simulink model "testing"  (R2025b)
settings: Solver=FixedStepDiscrete  StartTime=0.0  StopTime=20  RelTol=1e-3
InitFcn:
  | mcb_pmsm_foc_qep_f28379d_SIUnit_data
values from neighbouring files (symbols this model uses):
  A = [ -Rs/L,           0,                  0 ... (first row only)    [mcb_pmsm_fsfb_f28379d_param.m]    (also in v0_pmsm_fsfb_sim_for_flipsky_.m = [; v1_0_3_sim_param_fsfc.m = [)
  inverter = mcb.updateInverterParameters(pmsm,inverter,target)    [mcb_pmsm_foc_qep_f28379d_SIUnit_data.m]
  K = Ka_fsfb(1)    [mcb_pmsm_foc_qep_f28379d_SIUnit_data.m]    (also in mcb_pmsm_fsfb_f28379d_param.m = place(Ai, Bi, desired_poles); v0_pmsm_fsfb_sim_for_flipsky_.m = place(Ai, Bi, desired_poles); v1_0_3_sim_param_fsfc.m = place(Ai, Bi, desired_poles))
  Ki = -Ka_fsfb(2)    [mcb_pmsm_foc_qep_f28379d_SIUnit_data.m]    (also in mcb_pmsm_fsfb_f28379d_param.m = -K(:, n+1:end); v0_pmsm_fsfb_sim_for_flipsky_.m = -K(:, n+1:end); v1_0_3_sim_param_fsfc.m = -K(:, n+1:end))
  lambda_pm = pmsm.FluxPM    [mcb_pmsm_foc_qep_f28379d_SIUnit_data.m]
  PI_params = mcb.calcFOCGains(motor,Ts,Ts_speed,SpdLPFltCoeff=LPFltCoeff)    [mcb_pmsm_foc_qep_f28379d_SIUnit_data.m]
  pmsm = mcb.getPMSMParameters('Teknic2310P')    [mcb_pmsm_foc_qep_f28379d_SIUnit_data.m]
  Speed_Ki_Ts = Kis * Ts_speed    [mcb_pmsm_foc_qep_f28379d_SIUnit_data.m]
  Speed_Kp = Ks    [mcb_pmsm_foc_qep_f28379d_SIUnit_data.m]
  T_pwm = 1/PWM_frequency    (= 5e-05)    [mcb_pmsm_foc_qep_f28379d_SIUnit_data.m]
  target = mcb.getProcessorParameters('F28379D',PWM_frequency)    [mcb_pmsm_foc_qep_f28379d_SIUnit_data.m]
  Ts = T_pwm    (= 5e-05)    [mcb_pmsm_foc_qep_f28379d_SIUnit_data.m]    (also in v0_pmsm_fsfb_sim_for_flipsky_.m = 0.0001; v1_0_3_sim_param_fsfc.m = 0.0001)
  Ts_inverter = T_pwm/2    (= 2.5e-05)    [mcb_pmsm_foc_qep_f28379d_SIUnit_data.m]
  Ts_motor = T_pwm/2    (= 2.5e-05)    [mcb_pmsm_foc_qep_f28379d_SIUnit_data.m]
  Ts_simulink = T_pwm/2    (= 2.5e-05)    [mcb_pmsm_foc_qep_f28379d_SIUnit_data.m]
  Ts_speed = 10*Ts    (= 0.0005)    [mcb_pmsm_foc_qep_f28379d_SIUnit_data.m]
undefined symbols (not defined in the file or in its folder): bit, DiscIntNeverNeededParam, Down, GPTRIP1SEL, GPTRIP2SEL, TZ1, TZ2, Up
libraries: mcbcontrolslib x10, c2802xlib x7, simulink x5, c2837xDlib x4, mcbeeMathTransformLib x3, c280xlib x3, mcbpositiondecoderlib x3, svdschedulerlib x1, autolibpmsmexterior x1, slpidlib x1
(part 2 of 2)

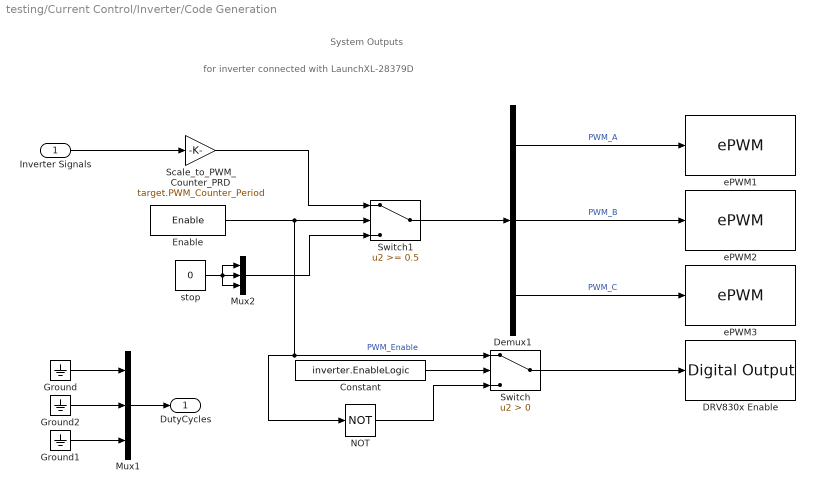
== system testing/Current Control/Inverter/Code Generation ==
  note: for inverter connected with LaunchXL-28379D
  note: System Outputs
  Inverter Signals : Inport
  Constant : Constant  Value=inverter.EnableLogic
  DRV830x Enable : c2837xDlib/Digital Output  GPIO_Number=GPIO120~GPIO127  GPIO_Bit0=off  GPIO_BIT0_Toggle=off  GPIO_Bit1=off  GPIO_BIT1_Toggle=off  GPIO_Bit2=off  GPIO_BIT2_Toggle=off  GPIO_Bit3=off  GPIO_BIT3_Toggle=off  GPIO_Bit4=on  GPIO_BIT4_Toggle=off  GPIO_Bit5=off  GPIO_BIT5_Toggle=off  GPIO_Bit6=off  GPIO_BIT6_Toggle=off  GPIO_Bit7=off  GPIO_BIT7_Toggle=off
  Demux1 : Demux  Outputs=3
  Enable : DataStoreRead  DataStoreName=Enable  IndexOptions=Index vector (dialog)  Indices=1  OutputSizes=1
  Ground : Ground
  Ground1 : Ground
  Ground2 : Ground
  Mux1 : Mux  Inputs=3
  Mux2 : Mux  Inputs=3
  NOT : Logic  Operator=NOT  IconShape=distinctive  AllPortsSameDT=off  OutDataTypeStr=boolean
  Scale_to_PWM_Counter_PRD : Gain  Gain=target.PWM_Counter_Period  OutDataTypeStr=uint16  RndMeth=Simplest
  Switch : Switch  Criteria=u2 > Threshold  SaturateOnIntegerOverflow=off  InputSameDT=off
  Switch1 : Switch  Threshold=0.5  SaturateOnIntegerOverflow=off  InputSameDT=off
  ePWM1 : c2802xlib/ePWM  PwmType=C2000_Type4  useModule=ePWM1  ePWMxLINKTBPRD=Not Linked  periodUnits=Clock cycles  timerSource=Specify via dialog  timerPeriod_clk=target.PWM_Counter_Period  timerPeriod_sec=0.0001  tbshadow=Counter equals to zero  countingMode=Up-Down  phaseActiveEnable=Disable  phaseDirection=Count down after sync  phaseActive=0  synchronizationEnable=off  dcaevt1Sync=off  dcbevt1Sync=off  synchronizationOption=Counter equals to zero (CTR=Zero)  dcbevt1SyncOut=off  dcaevt1SyncOut=off  cmpdSyncOut=off  cmpcSyncOut=off  cmpbSyncOut=off  zeroSyncOut=on  swfSyncOut=off  perSynchronizationOption=Counter equals to period (CTR=PRD)  clockPrescale=1  HSclockPrescale=1  enswap=off  ePWMxAStatus=on  ePWMxAactionLogic1=Do nothing  ePWMxAactionLogic2=Do nothing  ePWMxAactionLogic3=Clear  ePWMxAactionLogic4=Set  ePWMxAactionLogic5=Do nothing  ePWMxAactionLogic6=Do nothing  ePWMxACSFenable=off  ePWMxACSFvalue=Forcing disable  ePWMxASFreload=Zero  ePWMxBStatus=off  ePWMxBactionLogic1=Set  ePWMxBactionLogic2=Clear  ePWMxBactionLogic3=Do nothing  ePWMxBactionLogic4=Do nothing  ePWMxBactionLogic5=Clear  ePWMxBactionLogic6=Set  ePWMxBCSFenable=off  ePWMxBCSFvalue=Forcing disable  ePWMxBSFreload=Zero  ePWNxBOutWay=off  ePWMxLINKCMPA=Not Linked  CMPAUnits=Clock cycles  CMPASource=Input port  CMPAValue_per=50  CMPAValue_clk=floor(target.PWM_Counter_Period/2+1)  enCMPAshadow=Counter equals to zero (CTR=Zero)  ePWMxLINKCMPB=Not Linked  CMPBUnits=Clock cycles  CMPBSource=Specify via dialog  CMPBValue_per=50  CMPBValue_clk=floor(target.PWM_Counter_Period/2+1)  enCMPBshadow=Counter equals to zero (CTR=Zero)  ePWMxLINKCMPC=Not Linked  CMPCUnits=Clock cycles  CMPCSource=Specify via dialog  CMPCValue_per=50  CMPCValue_clk=32000  enCMPCshadow=Counter equals to zero (CTR=Zero)  ePWMxLINKCMPD=Not Linked  CMPDUnits=Clock cycles  CMPDSource=Specify via dialog  CMPDValue_per=50  CMPDValue_clk=32000  enCMPDshadow=Counter equals to zero (CTR=Zero)  enableDBePWMxA=on  enableDBePWMxB=on  enhalfcycle=off  DBpolarity=Active high complementary (AHC)  DBedgeDelay=Positive  DBSource_ePWMxA=ePWMxA  DBSource_ePWMxB=ePWMxA  DBPeriodUnits=Clock cycles  DBperiodSource=Specify via dialog  REDperiod=15  FEDperiod=15  REDperiod_sec=0  FEDperiod_sec=0  LoadModeDBRED=Immediate without using shadow  LoadModeDBFED=Immediate without using shadow  adcstartModuleA=on  adcrequestEventA=First event  adcstartEventA=Digital Compare Module A Event 1 start of conversion (DCAEVT1.soc)  adcstartEventA_type2=Counter equals to period (CTR=PRD)  adcstartModuleB=off  adcrequestEventB=First event  adcstartEventB=Counter equals to zero (CTR=Zero)  adcstartEventB_type2=Counter equals to zero (CTR=Zero)  intEn=off  intPrd=First event  intSel=Counter equals to zero (CTR=Zero)  intSel_type2=Counter equals to zero (CTR=Zero)  hrpe=off  enHRPWM=off  HRPWM_LoadMode=Counter equals to period (CTR=PRD)  HRPWM_CTLMode=Duty or Period control mode  HRPWM_EDGMode=Both edge  hrpeb=off  enHRPWMB=off  HRPWM_LoadModeB=Counter equals to zero (CTR=ZERO)  HRPWM_CTLModeB=Duty or Period control mode  HRPWM_EDGModeB=Both edge  enHRDBRED=off  enHRDBFED=off  enSFO=on  enautoconv=on  chopperEnable=off  chopperFrequency=1  chopperFirstwidth=1  chopperDuty=12.5%  tripZonesource=Specify via dialog  tzselOSHT1=off  tzselOSHT2=off  tzselOSHT3=off  tzselOSHT4=off  tzselOSHT5=off  tzselOSHT6=off  tzselOSHDCAEV1=off  tzselOSHDCBEV1=off  tzselCBC1=off  tzselCBC2=off  tzselCBC3=off  tzselCBC4=off  tzselCBC5=off  tzselCBC6=off  tzselCBCDCAEV2=off  tzselCBCDCBEV2=off  enTzOstIntr=off  enTzCbcIntr=off  enTzDCAEVT1Intr=off  enTzDCAEVT2Intr=off  enTzDCBEVT1Intr=off  enTzDCBEVT2Intr=off  tzclrCBCLatch=Counter equals to zero (CTR=Zero)  ePWMxAforced=No action  ePWMxBforced=No action  DCAEVT1forced=No action  DCBEVT1forced=No action  DCAEVT2forced=No action  DCBEVT2forced=No action  dcah=Trip Zone 1 input (TZ1)  dcal=Trip Zone 2 input (TZ2)  dcbh=Trip Zone 1 input (TZ1)  dcbl=Trip Zone 2 input (TZ2)  dcah_type2=GPTRIP1SEL/(TZ1)  dcal_type2=GPTRIP2SEL/(TZ2)  dcbh_type2=GPTRIP1SEL/(TZ1)  dcbl_type2=GPTRIP2SEL/(TZ2)  gendcaevt1=Event disabled  gendcaevt2=Event disabled  gendcbevt1=Event disabled  gendcbevt2=Event disabled  dcaevt1src=DCAEVT1 with sync  dcaevt2src=DCAEVT2 with sync  dcbevt1src=DCBEVT1 with sync  dcbevt2src=DCBEVT2 with sync  pulsesel=Counter equals to zero (CTR=Zero)  blankinv=off  blankoffset=0  blankwidth=0  evsrcsel=Filtered version of DCAEVT1 (DCAEVT1FILT)  encape=off
  ePWM2 : c2802xlib/ePWM  PwmType=C2000_Type4  useModule=ePWM2  ePWMxLINKTBPRD=Not Linked  periodUnits=Clock cycles  timerSource=Specify via dialog  timerPeriod_clk=target.PWM_Counter_Period  timerPeriod_sec=0.0001  tbshadow=Counter equals to zero  countingMode=Up-Down  phaseActiveEnable=Set counter to phase value specified via dialog  phaseDirection=Count up after sync  phaseActive=0  synchronizationEnable=off  dcaevt1Sync=off  dcbevt1Sync=off  synchronizationOption=Pass through (EPWMxSYNCI or SWFSYNC)  dcbevt1SyncOut=off  dcaevt1SyncOut=off  cmpdSyncOut=off  cmpcSyncOut=off  cmpbSyncOut=off  zeroSyncOut=off  swfSyncOut=on  perSynchronizationOption=Counter equals to period (CTR=PRD)  clockPrescale=1  HSclockPrescale=1  enswap=off  ePWMxAStatus=on  ePWMxAactionLogic1=Do nothing  ePWMxAactionLogic2=Do nothing  ePWMxAactionLogic3=Clear  ePWMxAactionLogic4=Set  ePWMxAactionLogic5=Do nothing  ePWMxAactionLogic6=Do nothing  ePWMxACSFenable=off  ePWMxACSFvalue=Forcing disable  ePWMxASFreload=Zero  ePWMxBStatus=off  ePWMxBactionLogic1=Set  ePWMxBactionLogic2=Clear  ePWMxBactionLogic3=Do nothing  ePWMxBactionLogic4=Do nothing  ePWMxBactionLogic5=Clear  ePWMxBactionLogic6=Set  ePWMxBCSFenable=off  ePWMxBCSFvalue=Forcing disable  ePWMxBSFreload=Zero  ePWNxBOutWay=off  ePWMxLINKCMPA=Not Linked  CMPAUnits=Clock cycles  CMPASource=Input port  CMPAValue_per=50  CMPAValue_clk=floor(target.PWM_Counter_Period/2+1)  enCMPAshadow=Counter equals to zero (CTR=Zero)  ePWMxLINKCMPB=Not Linked  CMPBUnits=Clock cycles  CMPBSource=Specify via dialog  CMPBValue_per=50  CMPBValue_clk=floor(target.PWM_Counter_Period/2+1)  enCMPBshadow=Counter equals to zero (CTR=Zero)  ePWMxLINKCMPC=Not Linked  CMPCUnits=Clock cycles  CMPCSource=Specify via dialog  CMPCValue_per=50  CMPCValue_clk=32000  enCMPCshadow=Counter equals to zero (CTR=Zero)  ePWMxLINKCMPD=Not Linked  CMPDUnits=Clock cycles  CMPDSource=Specify via dialog  CMPDValue_per=50  CMPDValue_clk=32000  enCMPDshadow=Counter equals to zero (CTR=Zero)  enableDBePWMxA=on  enableDBePWMxB=on  enhalfcycle=off  DBpolarity=Active high complementary (AHC)  DBedgeDelay=Positive  DBSource_ePWMxA=ePWMxA  DBSource_ePWMxB=ePWMxA  DBPeriodUnits=Clock cycles  DBperiodSource=Specify via dialog  REDperiod=15  FEDperiod=15  REDperiod_sec=0  FEDperiod_sec=0  LoadModeDBRED=Immediate without using shadow  LoadModeDBFED=Immediate without using shadow  adcstartModuleA=off  adcrequestEventA=First event  adcstartEventA=Digital Compare Module A Event 1 start of conversion (DCAEVT1.soc)  adcstartEventA_type2=Counter equals to period (CTR=PRD)  adcstartModuleB=off  adcrequestEventB=First event  adcstartEventB=Counter equals to zero (CTR=Zero)  adcstartEventB_type2=Counter equals to zero (CTR=Zero)  intEn=off  intPrd=First event  intSel=Counter equals to zero (CTR=Zero)  intSel_type2=Counter equals to zero (CTR=Zero)  hrpe=off  enHRPWM=off  HRPWM_LoadMode=Counter equals to period (CTR=PRD)  HRPWM_CTLMode=Duty or Period control mode  HRPWM_EDGMode=Both edge  hrpeb=off  enHRPWMB=off  HRPWM_LoadModeB=Counter equals to zero (CTR=ZERO)  HRPWM_CTLModeB=Duty or Period control mode  HRPWM_EDGModeB=Both edge  enHRDBRED=off  enHRDBFED=off  enSFO=on  enautoconv=on  chopperEnable=off  chopperFrequency=1  chopperFirstwidth=1  chopperDuty=12.5%  tripZonesource=Specify via dialog  tzselOSHT1=off  tzselOSHT2=off  tzselOSHT3=off  tzselOSHT4=off  tzselOSHT5=off  tzselOSHT6=off  tzselOSHDCAEV1=off  tzselOSHDCBEV1=off  tzselCBC1=off  tzselCBC2=off  tzselCBC3=off  tzselCBC4=off  tzselCBC5=off  tzselCBC6=off  tzselCBCDCAEV2=off  tzselCBCDCBEV2=off  enTzOstIntr=off  enTzCbcIntr=off  enTzDCAEVT1Intr=off  enTzDCAEVT2Intr=off  enTzDCBEVT1Intr=off  enTzDCBEVT2Intr=off  tzclrCBCLatch=Counter equals to zero (CTR=Zero)  ePWMxAforced=No action  ePWMxBforced=No action  DCAEVT1forced=No action  DCBEVT1forced=No action  DCAEVT2forced=No action  DCBEVT2forced=No action  dcah=Trip Zone 1 input (TZ1)  dcal=Trip Zone 2 input (TZ2)  dcbh=Trip Zone 1 input (TZ1)  dcbl=Trip Zone 2 input (TZ2)  dcah_type2=GPTRIP1SEL/(TZ1)  dcal_type2=GPTRIP2SEL/(TZ2)  dcbh_type2=GPTRIP1SEL/(TZ1)  dcbl_type2=GPTRIP2SEL/(TZ2)  gendcaevt1=Event disabled  gendcaevt2=Event disabled  gendcbevt1=Event disabled  gendcbevt2=Event disabled  dcaevt1src=DCAEVT1 with sync  dcaevt2src=DCAEVT2 with sync  dcbevt1src=DCBEVT1 with sync  dcbevt2src=DCBEVT2 with sync  pulsesel=Counter equals to zero (CTR=Zero)  blankinv=off  blankoffset=0  blankwidth=0  evsrcsel=Filtered version of DCAEVT1 (DCAEVT1FILT)  encape=off
  ePWM3 : c2802xlib/ePWM  PwmType=C2000_Type4  useModule=ePWM3  ePWMxLINKTBPRD=Not Linked  periodUnits=Clock cycles  timerSource=Specify via dialog  timerPeriod_clk=target.PWM_Counter_Period  timerPeriod_sec=0.0001  tbshadow=Counter equals to zero  countingMode=Up-Down  phaseActiveEnable=Set counter to phase value specified via dialog  phaseDirection=Count up after sync  phaseActive=0  synchronizationEnable=off  dcaevt1Sync=off  dcbevt1Sync=off  synchronizationOption=Pass through (EPWMxSYNCI or SWFSYNC)  dcbevt1SyncOut=off  dcaevt1SyncOut=off  cmpdSyncOut=off  cmpcSyncOut=off  cmpbSyncOut=off  zeroSyncOut=off  swfSyncOut=on  perSynchronizationOption=Counter equals to period (CTR=PRD)  clockPrescale=1  HSclockPrescale=1  enswap=off  ePWMxAStatus=on  ePWMxAactionLogic1=Do nothing  ePWMxAactionLogic2=Do nothing  ePWMxAactionLogic3=Clear  ePWMxAactionLogic4=Set  ePWMxAactionLogic5=Do nothing  ePWMxAactionLogic6=Do nothing  ePWMxACSFenable=off  ePWMxACSFvalue=Forcing disable  ePWMxASFreload=Zero  ePWMxBStatus=off  ePWMxBactionLogic1=Set  ePWMxBactionLogic2=Clear  ePWMxBactionLogic3=Do nothing  ePWMxBactionLogic4=Do nothing  ePWMxBactionLogic5=Clear  ePWMxBactionLogic6=Set  ePWMxBCSFenable=off  ePWMxBCSFvalue=Forcing disable  ePWMxBSFreload=Zero  ePWNxBOutWay=off  ePWMxLINKCMPA=Not Linked  CMPAUnits=Clock cycles  CMPASource=Input port  CMPAValue_per=50  CMPAValue_clk=floor(target.PWM_Counter_Period/2+1)  enCMPAshadow=Counter equals to zero (CTR=Zero)  ePWMxLINKCMPB=Not Linked  CMPBUnits=Clock cycles  CMPBSource=Specify via dialog  CMPBValue_per=50  CMPBValue_clk=floor(target.PWM_Counter_Period/2+1)  enCMPBshadow=Counter equals to zero (CTR=Zero)  ePWMxLINKCMPC=Not Linked  CMPCUnits=Clock cycles  CMPCSource=Specify via dialog  CMPCValue_per=50  CMPCValue_clk=32000  enCMPCshadow=Counter equals to zero (CTR=Zero)  ePWMxLINKCMPD=Not Linked  CMPDUnits=Clock cycles  CMPDSource=Specify via dialog  CMPDValue_per=50  CMPDValue_clk=32000  enCMPDshadow=Counter equals to zero (CTR=Zero)  enableDBePWMxA=on  enableDBePWMxB=on  enhalfcycle=off  DBpolarity=Active high complementary (AHC)  DBedgeDelay=Positive  DBSource_ePWMxA=ePWMxA  DBSource_ePWMxB=ePWMxA  DBPeriodUnits=Clock cycles  DBperiodSource=Specify via dialog  REDperiod=15  FEDperiod=15  REDperiod_sec=0  FEDperiod_sec=0  LoadModeDBRED=Immediate without using shadow  LoadModeDBFED=Immediate without using shadow  adcstartModuleA=off  adcrequestEventA=First event  adcstartEventA=Digital Compare Module A Event 1 start of conversion (DCAEVT1.soc)  adcstartEventA_type2=Counter equals to period (CTR=PRD)  adcstartModuleB=off  adcrequestEventB=First event  adcstartEventB=Counter equals to zero (CTR=Zero)  adcstartEventB_type2=Counter equals to zero (CTR=Zero)  intEn=off  intPrd=First event  intSel=Counter equals to zero (CTR=Zero)  intSel_type2=Counter equals to zero (CTR=Zero)  hrpe=off  enHRPWM=off  HRPWM_LoadMode=Counter equals to period (CTR=PRD)  HRPWM_CTLMode=Duty or Period control mode  HRPWM_EDGMode=Both edge  hrpeb=off  enHRPWMB=off  HRPWM_LoadModeB=Counter equals to zero (CTR=ZERO)  HRPWM_CTLModeB=Duty or Period control mode  HRPWM_EDGModeB=Both edge  enHRDBRED=off  enHRDBFED=off  enSFO=on  enautoconv=on  chopperEnable=off  chopperFrequency=1  chopperFirstwidth=1  chopperDuty=12.5%  tripZonesource=Specify via dialog  tzselOSHT1=off  tzselOSHT2=off  tzselOSHT3=off  tzselOSHT4=off  tzselOSHT5=off  tzselOSHT6=off  tzselOSHDCAEV1=off  tzselOSHDCBEV1=off  tzselCBC1=off  tzselCBC2=off  tzselCBC3=off  tzselCBC4=off  tzselCBC5=off  tzselCBC6=off  tzselCBCDCAEV2=off  tzselCBCDCBEV2=off  enTzOstIntr=off  enTzCbcIntr=off  enTzDCAEVT1Intr=off  enTzDCAEVT2Intr=off  enTzDCBEVT1Intr=off  enTzDCBEVT2Intr=off  tzclrCBCLatch=Counter equals to zero (CTR=Zero)  ePWMxAforced=No action  ePWMxBforced=No action  DCAEVT1forced=No action  DCBEVT1forced=No action  DCAEVT2forced=No action  DCBEVT2forced=No action  dcah=Trip Zone 1 input (TZ1)  dcal=Trip Zone 2 input (TZ2)  dcbh=Trip Zone 1 input (TZ1)  dcbl=Trip Zone 2 input (TZ2)  dcah_type2=GPTRIP1SEL/(TZ1)  dcal_type2=GPTRIP2SEL/(TZ2)  dcbh_type2=GPTRIP1SEL/(TZ1)  dcbl_type2=GPTRIP2SEL/(TZ2)  gendcaevt1=Event disabled  gendcaevt2=Event disabled  gendcbevt1=Event disabled  gendcbevt2=Event disabled  dcaevt1src=DCAEVT1 with sync  dcaevt2src=DCAEVT2 with sync  dcbevt1src=DCBEVT1 with sync  dcbevt2src=DCBEVT2 with sync  pulsesel=Counter equals to zero (CTR=Zero)  blankinv=off  blankoffset=0  blankwidth=0  evsrcsel=Filtered version of DCAEVT1 (DCAEVT1FILT)  encape=off
  stop : Constant  Value=0  OutDataTypeStr=uint16
  DutyCycles : Outport  VectorParamsAs1DForOutWhenUnconnected=off
  wires:
  Demux1/3 -> ePWM3/1  "PWM_C"
  Scale_to_PWM_Counter_PRD/1 -> Switch1/1
  Mux2/1 -> Switch1/3
  stop/1 -> Mux2/3, Mux2/2, Mux2/1
  Enable/1 -> NOT/1, Switch/1, Switch1/2  "PWM_Enable"
  Demux1/2 -> ePWM2/1  "PWM_B"
  Switch1/1 -> Demux1/1
  Demux1/1 -> ePWM1/1  "PWM_A"
  Inverter Signals/1 -> Scale_to_PWM_Counter_PRD/1
  Ground/1 -> Mux1/1
  Ground1/1 -> Mux1/3
  Ground2/1 -> Mux1/2
  Mux1/1 -> DutyCycles/1
  Switch/1 -> DRV830x Enable/1
  NOT/1 -> Switch/3
  Constant/1 -> Switch/2

== system testing/Current Control/Inverter/Simulation ==
  Inverter Signals : Inport
  Data Type Duplicate : DataTypeDuplicate
  Enable : DataStoreRead  DataStoreName=Enable  IndexOptions=Index vector (dialog)  Indices=1  OutputSizes=1
  Mux2 : Mux  Inputs=3
  Switch1 : Switch  Threshold=0.5  RndMeth=Simplest  SaturateOnIntegerOverflow=off  InputSameDT=off
  stop : Constant  Value=0  OutDataTypeStr=Inherit: Inherit via back propagation
  DutyCycles : Outport  VectorParamsAs1DForOutWhenUnconnected=off
  wires:
  stop/1 -> Data Type Duplicate/2, Mux2/1, Mux2/3, Mux2/2
  Mux2/1 -> Switch1/3
  Switch1/1 -> DutyCycles/1
  Inverter Signals/1 -> Data Type Duplicate/1, Switch1/1  "PWM Duty Cycles"
  Enable/1 -> Switch1/2  "PWM_Enable"

== system testing/Hardware Init/Variant Subsystem/Code Generation ==
  note: for BoostXL-DRV8305 connected to LaunchXL-28379D
  note: System Outputs
  note: Enable ADC offset calibration only when motor is not loaded and not rotating due to external factors
  In1 : Inport
  ADC Calibration Enable : Constant  Value=inverter.ADCOffsetCalibEnable
  "Calculate ADC Offset " : Subsystem  Priority=1001  TreatAsAtomicUnit=on
  DRV Enable : Subsystem  Priority=1
  Default ADC Offset : Subsystem  Priority=1001  TreatAsAtomicUnit=on
  NOT : Logic  Operator=NOT  IconShape=distinctive  AllPortsSameDT=off  OutDataTypeStr=boolean
  wires:
  In1/1 -> DRV Enable/1(In)
  NOT/1 -> Default ADC Offset/Enable
  ADC Calibration Enable/1 -> NOT/1, "Calculate ADC Offset "/Enable

== system testing/Hardware Init/Variant Subsystem/Simulation ==
  In1 : Inport
  Terminator : Terminator
  wires:
  In1/1 -> Terminator/1

== system testing/Heartbeat LED/Heartbeat LED/Code generation ==
  In1 : Inport
  Digital Output : c2837xDlib/Digital Output  GPIO_Number=GPIO32~GPIO39  GPIO_Bit0=off  GPIO_BIT0_Toggle=on  GPIO_Bit1=off  GPIO_BIT1_Toggle=off  GPIO_Bit2=on  GPIO_BIT2_Toggle=on  GPIO_Bit3=off  GPIO_BIT3_Toggle=off  GPIO_Bit4=off  GPIO_BIT4_Toggle=off  GPIO_Bit5=off  GPIO_BIT5_Toggle=off  GPIO_Bit6=off  GPIO_BIT6_Toggle=off  GPIO_Bit7=off  GPIO_BIT7_Toggle=off
  wires:
  In1/1 -> Digital Output/1

== system testing/Heartbeat LED/Heartbeat LED/Simulation ==
  In1 : Inport
  Simulation_Terminator : Terminator
  wires:
  In1/1 -> Simulation_Terminator/1

== system testing/Inverter and Motor - Plant Model/Simulation/Inverter ==
  Duty_abc : Inport
  Average_Value_Inverter : Subsystem
  Constant2 : Constant  Value=inverter.V_dc  OutDataTypeStr=single  SampleTime=-1
  Data Type Conversion1 : DataTypeConversion  OutDataTypeStr=single  RndMeth=Simplest  SaturateOnIntegerOverflow=off
  Demux : Demux  Outputs=3
  Inverter_delay : DiscreteTransferFcn  Numerator=[1-exp(-Ts_inverter/(T_pwm/2))]  Denominator=[1 -exp(-Ts_inverter/(T_pwm/2))]  RndMeth=Simplest
  Mux : Mux  Inputs=3
  Rate Transition3 : RateTransition  Integrity=off  OutPortSampleTime=Ts_inverter
  Vabc : Outport  VectorParamsAs1DForOutWhenUnconnected=off
  wires:
  Average_Value_Inverter/2(Vb) -> Mux/2
  Mux/1 -> Inverter_delay/1
  Constant2/1 -> Average_Value_Inverter/4(Vdc)
  Average_Value_Inverter/3(Vc) -> Mux/3
  Average_Value_Inverter/1(Va) -> Mux/1
  Demux/1 -> Average_Value_Inverter/1(Vao)
  Demux/3 -> Average_Value_Inverter/3(Vco)
  Demux/2 -> Average_Value_Inverter/2(Vbo)
  Data Type Conversion1/1 -> Rate Transition3/1
  Rate Transition3/1 -> Demux/1
  Inverter_delay/1 -> Vabc/1
  Duty_abc/1 -> Data Type Conversion1/1

== system testing/Inverter and Motor - Plant Model/Simulation/Load_Profile (Torque) ==
  Data Type Conversion : DataTypeConversion  OutDataTypeStr=single  SaturateOnIntegerOverflow=off  RndMeth=Floor
  IIR Filter : mcbcontrolslib/IIR Filter  VariantControl=Low Pass Filter  VariantSelect=Low-pass  FilterConstantInputType=Specify via dialog  Filter_constant=0.01  InitialOutput=Specify via dialog  InitialOutputValue=0  ExternalReset=none  advancedSettings=off  Ts=50e-6  cutOff_freq=32.1525
  T_load : Step  Time=2  Before=0.05*pmsm.T_rated  After=0.5*pmsm.T_rated  SampleTime=Ts_simulink
  Load_Trq : Outport  VectorParamsAs1DForOutWhenUnconnected=off
  wires:
  Data Type Conversion/1 -> IIR Filter/1
  T_load/1 -> Data Type Conversion/1
  IIR Filter/1 -> Load_Trq/1

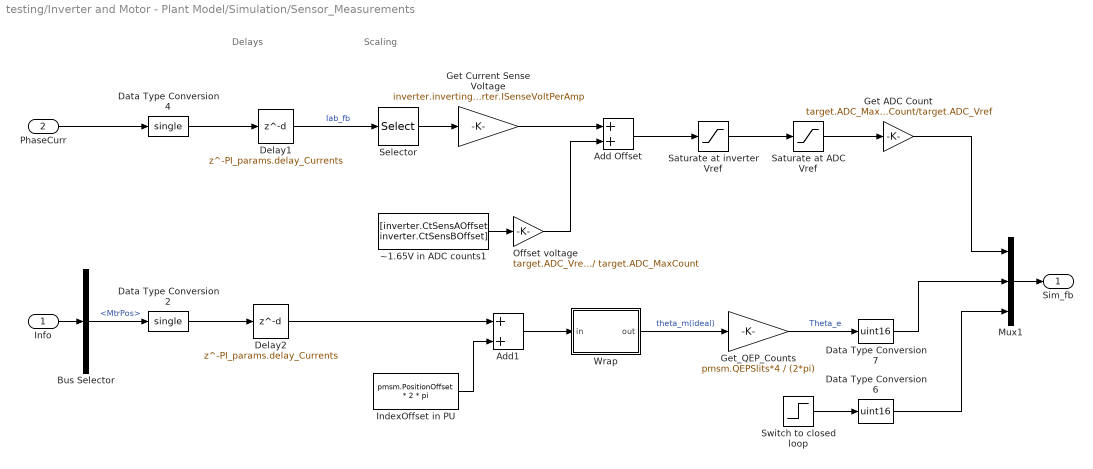
== system testing/Inverter and Motor - Plant Model/Simulation/Sensor_Measurements ==
  note: Scaling
  note: Delays
  Info : Inport
  PhaseCurr : Inport  Port=2
  Add Offset : Sum  RndMeth=Simplest
  Add1 : Sum  RndMeth=Simplest
  Bus Selector : BusSelector  OutputSignals=MtrPos
  Data Type Conversion2 : DataTypeConversion  OutDataTypeStr=single  RndMeth=Simplest  SaturateOnIntegerOverflow=off
  Data Type Conversion4 : DataTypeConversion  OutDataTypeStr=single  RndMeth=Simplest  SaturateOnIntegerOverflow=off
  Data Type Conversion6 : DataTypeConversion  OutDataTypeStr=uint16  RndMeth=Simplest  SaturateOnIntegerOverflow=off
  Data Type Conversion7 : DataTypeConversion  OutDataTypeStr=uint16  RndMeth=Simplest  SaturateOnIntegerOverflow=off
  Delay1 : Delay  DelayLength=PI_params.delay_Currents
  Delay2 : Delay  DelayLength=PI_params.delay_Currents
  Get ADC Count : Gain  Gain=target.ADC_MaxCount/target.ADC_Vref  OutMin=0  OutMax=target.ADC_MaxCount  OutDataTypeStr=uint16  RndMeth=Simplest
  Get Current Sense Voltage : Gain  Gain=inverter.invertingAmp * inverter.ISenseVoltPerAmp  RndMeth=Simplest  OutDataTypeStr=Inherit: Same as input
  Get_QEP_Counts : Gain  Gain=pmsm.QEPSlits*4 / (2*pi)  OutDataTypeStr=uint16  RndMeth=Simplest
  IndexOffset in PU : Constant  Value=pmsm.PositionOffset * 2 * pi  OutDataTypeStr=single  SampleTime=-1
  Mux1 : Mux  Inputs=3
  Offset voltage : Gain  Gain=target.ADC_Vref / target.ADC_MaxCount  RndMeth=Simplest
  Saturate at ADC Vref : Saturate  UpperLimit=target.ADC_Vref  LowerLimit=0
  Saturate at inverter Vref : Saturate  UpperLimit=inverter.ISenseVref  LowerLimit=0
  Selector : Selector  InputPortWidth=3  IndexOptions=Index vector (dialog)  Indices=[1 2]  OutputSizes=1
  Switch to closed loop : Step  Time=0.1  SampleTime=Ts_motor
  Wrap : Subsystem
  ~1.65V in ADC counts1 : Constant  Value=[inverter.CtSensAOffset inverter.CtSensBOffset]  OutDataTypeStr=uint16  SampleTime=-1
  Sim_fb : Outport  VectorParamsAs1DForOutWhenUnconnected=off
  wires:
  Delay1/1 -> Selector/1  "Iab_fb"
  Data Type Conversion4/1 -> Delay1/1
  PhaseCurr/1 -> Data Type Conversion4/1
  Info/1 -> Bus Selector/1
  Bus Selector/1 -> Data Type Conversion2/1  "<MtrPos>"
  Data Type Conversion2/1 -> Delay2/1
  Mux1/1 -> Sim_fb/1
  Delay2/1 -> Add1/1
  IndexOffset in PU/1 -> Add1/2
  Add1/1 -> Wrap/1(in)
  Get_QEP_Counts/1 -> Data Type Conversion7/1  "Theta_e"
  Wrap/1(out) -> Get_QEP_Counts/1  "theta_m(ideal)"
  Switch to closed loop/1 -> Data Type Conversion6/1
  ~1.65V in ADC counts1/1 -> Offset voltage/1
  Get Current Sense Voltage/1 -> Add Offset/1
  Saturate at ADC Vref/1 -> Get ADC Count/1
  Add Offset/1 -> Saturate at inverter Vref/1
  Saturate at inverter Vref/1 -> Saturate at ADC Vref/1
  Selector/1 -> Get Current Sense Voltage/1
  Offset voltage/1 -> Add Offset/2
  Data Type Conversion6/1 -> Mux1/3
  Data Type Conversion7/1 -> Mux1/2
  Get ADC Count/1 -> Mux1/1

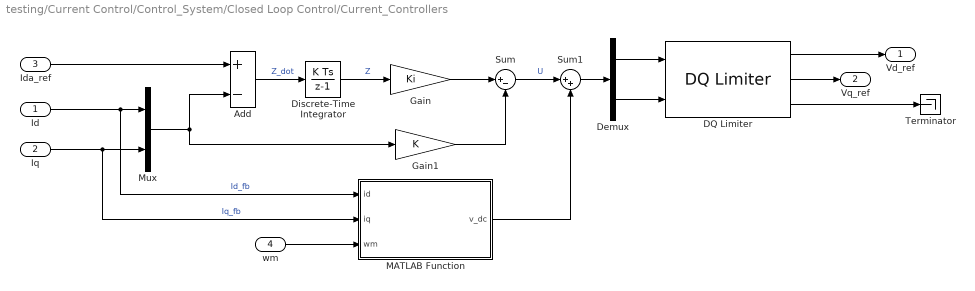
== system testing/Current Control/Control_System/Closed Loop Control/Current_Controllers ==
  Id : Inport
  Iq : Inport  Port=2
  Ida_ref : Inport  Port=3
  wm : Inport  Port=4
  Add : Sum  Inputs=+-
  DQ Limiter : mcbcontrolslib/DQ Limiter  satMethodInputType=Specify via dialog  satMethodSelected=D-Q equivalence  satLimitInputType=Specify via dialog  Vmax=inverter.V_dc/sqrt(3) *0.95
  Demux : Demux  Outputs=2
  Discrete-Time Integrator : DiscreteIntegrator  SampleTime=-1  ICPrevOutput=DiscIntNeverNeededParam  ICPrevScaledInput=DiscIntNeverNeededParam
  Gain : Gain  Gain=Ki
  Gain1 : Gain  Gain=K
  MATLAB Function : MATLAB Function  TreatAsAtomicUnit=on
  Mux : Mux  Inputs=2
  Sum : Sum  Inputs=|+-
  Sum1 : Sum  Inputs=|++
  Terminator : Terminator
  Vd_ref : Outport  VectorParamsAs1DForOutWhenUnconnected=off
  Vq_ref : Outport  Port=2  VectorParamsAs1DForOutWhenUnconnected=off
  wires:
  Ida_ref/1 -> Add/1
  Demux/1 -> DQ Limiter/1
  Demux/2 -> DQ Limiter/2
  DQ Limiter/2 -> Vq_ref/1
  DQ Limiter/1 -> Vd_ref/1
  DQ Limiter/3 -> Terminator/1
  Id/1 -> MATLAB Function/1(id), Mux/1  "Id_fb"
  Iq/1 -> MATLAB Function/2(iq), Mux/2  "Iq_fb"
  Mux/1 -> Gain1/1, Add/2
  Add/1 -> Discrete-Time Integrator/1  "Z_dot"
  Discrete-Time Integrator/1 -> Gain/1  "Z"
  Gain/1 -> Sum/1
  Gain1/1 -> Sum/2
  MATLAB Function/1(v_dc) -> Sum1/2
  Sum/1 -> Sum1/1  "U"
  wm/1 -> MATLAB Function/3(wm)
  Sum1/1 -> Demux/1

== system testing/Current Control/Control_System/Closed Loop Control/SVPWM ==
  Va : Inport
  Vb : Inport  Port=2
  Constant : Constant  Value=0.5  OutDataTypeStr=dataType  SampleTime=-1
  Mux1 : Mux  Inputs=3
  Normalize [-0.5 to 0.5] : Gain  Gain=1/ (2 * inverter.V_dc / sqrt(3))  RndMeth=Simplest  OutDataTypeStr=Inherit: Same as input
  Space Vector Generator : mcbcontrolslib/PWM Reference Generator  inSignal=Valphabeta  modType=SVM: space vector modulation
  Sum : Sum  Inputs=|++
  Duty_abc : Outport
  wires:
  Mux1/1 -> Normalize [-0.5 to 0.5]/1
  Normalize [-0.5 to 0.5]/1 -> Sum/1
  Va/1 -> Space Vector Generator/1
  Space Vector Generator/1 -> Mux1/1
  Constant/1 -> Sum/2
  Space Vector Generator/3 -> Mux1/3
  Space Vector Generator/2 -> Mux1/2
  Vb/1 -> Space Vector Generator/2
  Sum/1 -> Duty_abc/1

== system testing/Current Control/Control_System/Open Loop Start-Up/Convert to Duty Cycles ==
  In : Inport
  Constant : Constant  Value=0.5  OutDataTypeStr=dataType  SampleTime=-1
  Normalize : Gain  Gain=1/2  RndMeth=Simplest  OutDataTypeStr=Inherit: Same as input
  Sum1 : Sum  Inputs=|++
  Out : Outport
  wires:
  Normalize/1 -> Sum1/1
  Constant/1 -> Sum1/2
  In/1 -> Normalize/1
  Sum1/1 -> Out/1

== system testing/Current Control/Control_System/Open Loop Start-Up/Ramp Generator ==
  Ramp_Time : Inport
  Enable : Inport  Port=2
  Divide : Product  Inputs=*/  RndMeth=Simplest  OutDataTypeStr=Inherit: Same as first input
  NOT : Logic  Operator=NOT  IconShape=distinctive  AllPortsSameDT=off  OutDataTypeStr=boolean
  One : Constant  OutDataTypeStr=dataType  SampleTime=-1
  Ramp Generator : DiscreteIntegrator  IntegratorMethod=Accumulation: Forward Euler  gainval=1  ExternalReset=sampled level  SampleTime=-1  OutDataTypeStr=dataType  RndMeth=Simplest  LimitOutput=on  UpperSaturationLimit=1  LowerSaturationLimit=0  ICPrevOutput=DiscIntNeverNeededParam  ICPrevScaledInput=DiscIntNeverNeededParam
  Sample_Time : Gain  Gain=Ts  RndMeth=Simplest  OutDataTypeStr=Inherit: Same as input
  Ramp : Outport
  wires:
  Divide/1 -> Sample_Time/1
  Ramp Generator/1 -> Ramp/1  "Eps"
  Sample_Time/1 -> Ramp Generator/1
  One/1 -> Divide/1
  Ramp_Time/1 -> Divide/2
  Enable/1 -> NOT/1
  NOT/1 -> Ramp Generator/2

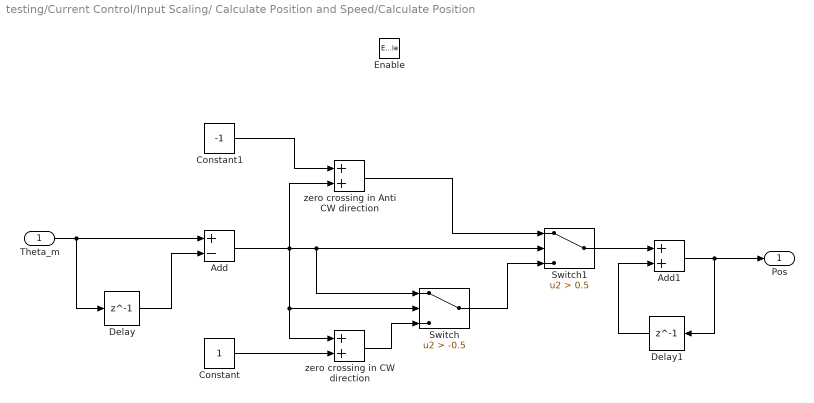
== system testing/Current Control/Input Scaling/ Calculate Position and Speed/Calculate Position ==
  Theta_m : Inport
  Enable : EnablePort
  Add : Sum  Inputs=+-
  Add1 : Sum
  Constant : Constant  OutDataTypeStr=dataType
  Constant1 : Constant  Value=-1  OutDataTypeStr=dataType
  Delay : Delay  DelayLength=1
  Delay1 : Delay  DelayLength=1
  Switch : Switch  Criteria=u2 > Threshold  Threshold=-0.5  SaturateOnIntegerOverflow=off  InputSameDT=off
  Switch1 : Switch  Criteria=u2 > Threshold  Threshold=0.5  SaturateOnIntegerOverflow=off  InputSameDT=off
  zero crossing in Anti CW direction : Sum
  zero crossing in CW direction : Sum
  Pos : Outport
  wires:
  Theta_m/1 -> Delay/1, Add/1
  Delay/1 -> Add/2
  Delay1/1 -> Add1/2
  Add1/1 -> Pos/1, Delay1/1
  Add/1 -> zero crossing in Anti CW direction/2, zero crossing in CW direction/1, Switch/2, Switch/1, Switch1/2
  zero crossing in CW direction/1 -> Switch/3
  Constant1/1 -> zero crossing in Anti CW direction/1
  zero crossing in Anti CW direction/1 -> Switch1/1
  Switch/1 -> Switch1/3
  Switch1/1 -> Add1/1
  Constant/1 -> zero crossing in CW direction/2

== system testing/Current Control/Input Scaling/ Calculate Position and Speed/IndexFinder ==
  In1 : Inport
  Enable : EnablePort
  AND : Logic  AllPortsSameDT=off  OutDataTypeStr=boolean
  Compare To Constant : simulink/Logic and Bit Operations/Compare To Constant  relop===  const=0  OutDataTypeStr=boolean
  Compare To Constant1 : simulink/Logic and Bit Operations/Compare To Constant  relop=>  const=0  OutDataTypeStr=boolean
  Delay3 : Delay  DelayLength=1
  Out1 : Outport
  wires:
  In1/1 -> Delay3/1, Compare To Constant1/1
  Compare To Constant1/1 -> AND/2
  Compare To Constant/1 -> AND/1
  Delay3/1 -> Compare To Constant/1
  AND/1 -> Out1/1

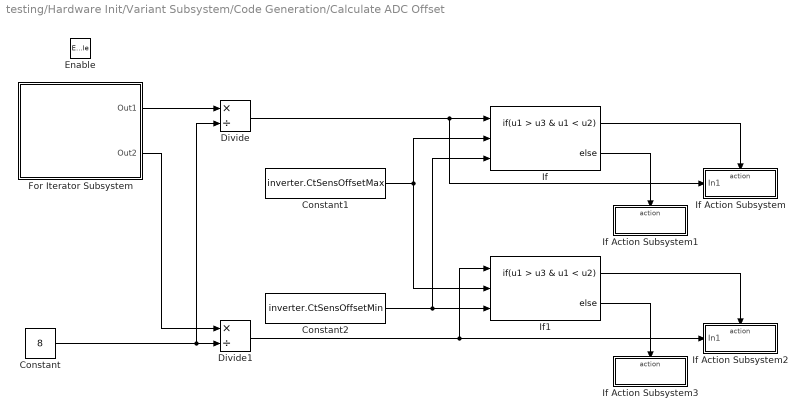
== system testing/Hardware Init/Variant Subsystem/Code Generation/Calculate ADC Offset  ==
  Enable : EnablePort
  Constant : Constant  Value=8
  Constant1 : Constant  Value=inverter.CtSensOffsetMax  OutDataTypeStr=Inherit: Inherit via back propagation
  Constant2 : Constant  Value=inverter.CtSensOffsetMin  OutDataTypeStr=Inherit: Inherit via back propagation
  Divide : Product  Inputs=*/  OutDataTypeStr=uint16
  Divide1 : Product  Inputs=*/  OutDataTypeStr=uint16
  For Iterator Subsystem : Subsystem  TreatAsAtomicUnit=on
  If : If  NumInputs=3  IfExpression=u1 > u3 & u1 < u2
  If Action Subsystem : Subsystem  TreatAsAtomicUnit=on
  If Action Subsystem1 : Subsystem  TreatAsAtomicUnit=on
  If Action Subsystem2 : Subsystem  TreatAsAtomicUnit=on
  If Action Subsystem3 : Subsystem  TreatAsAtomicUnit=on
  If1 : If  NumInputs=3  IfExpression=u1 > u3 & u1 < u2
  wires:
  For Iterator Subsystem/1(Out1) -> Divide/1
  If1/2 -> If Action Subsystem3/Action
  If1/1 -> If Action Subsystem2/Action
  Constant1/1 -> If/2, If1/2
  If/2 -> If Action Subsystem1/Action
  For Iterator Subsystem/2(Out2) -> Divide1/1
  If/1 -> If Action Subsystem/Action
  Constant2/1 -> If/3, If1/3
  Divide1/1 -> If Action Subsystem2/1(In1), If1/1
  Constant/1 -> Divide1/2, Divide/2
  Divide/1 -> If Action Subsystem/1(In1), If/1

== system testing/Hardware Init/Variant Subsystem/Code Generation/DRV Enable ==
  note: Enable Inverter
  In : Inport
  ADC Gain Setting : Subsystem
  Constant : Constant  Value=inverter.EnableLogic
  DRV830x Enable : Constant  OutDataTypeStr=uint16  SampleTime=-1
  Digital Output : c2837xDlib/Digital Output  Priority=10  GPIO_Number=GPIO120~GPIO127  GPIO_Bit0=off  GPIO_BIT0_Toggle=off  GPIO_Bit1=off  GPIO_BIT1_Toggle=off  GPIO_Bit2=off  GPIO_BIT2_Toggle=off  GPIO_Bit3=off  GPIO_BIT3_Toggle=off  GPIO_Bit4=on  GPIO_BIT4_Toggle=off  GPIO_Bit5=off  GPIO_BIT5_Toggle=off  GPIO_Bit6=off  GPIO_BIT6_Toggle=off  GPIO_Bit7=off  GPIO_BIT7_Toggle=off
  Digital Output1 : c2837xDlib/Digital Output  Priority=10  GPIO_Number=GPIO16~GPIO23  GPIO_Bit0=off  GPIO_BIT0_Toggle=off  GPIO_Bit1=off  GPIO_BIT1_Toggle=off  GPIO_Bit2=off  GPIO_BIT2_Toggle=off  GPIO_Bit3=off  GPIO_BIT3_Toggle=off  GPIO_Bit4=off  GPIO_BIT4_Toggle=off  GPIO_Bit5=off  GPIO_BIT5_Toggle=off  GPIO_Bit6=on  GPIO_BIT6_Toggle=off  GPIO_Bit7=off  GPIO_BIT7_Toggle=off
  NOT : Logic  Operator=NOT  IconShape=distinctive  AllPortsSameDT=off  OutDataTypeStr=boolean
  RunTimeMeasurement : Constant  OutDataTypeStr=uint16  SampleTime=-1
  Switch : Switch  Criteria=u2 > Threshold  SaturateOnIntegerOverflow=off  InputSameDT=off
  wires:
  RunTimeMeasurement/1 -> Digital Output1/1
  Switch/1 -> Digital Output/1
  DRV830x Enable/1 -> NOT/1, Switch/1
  NOT/1 -> Switch/3
  Constant/1 -> ADC Gain Setting/Enable, Switch/2
  In/1 -> ADC Gain Setting/1(In)

== system testing/Hardware Init/Variant Subsystem/Code Generation/Default ADC Offset ==
  Enable : EnablePort
  Constant : Constant  Value=inverter.CtSensAOffset  OutDataTypeStr=Inherit: Inherit via back propagation
  Constant1 : Constant  Value=inverter.CtSensBOffset  OutDataTypeStr=Inherit: Inherit via back propagation
  Data Store Write1 : DataStoreWrite  DataStoreName=IaOffset  IndexOptions=Index vector (dialog)  Indices=1  OutputSizes=1
  Data Store Write2 : DataStoreWrite  DataStoreName=IbOffset  IndexOptions=Index vector (dialog)  Indices=1  OutputSizes=1
  wires:
  Constant/1 -> Data Store Write1/1
  Constant1/1 -> Data Store Write2/1

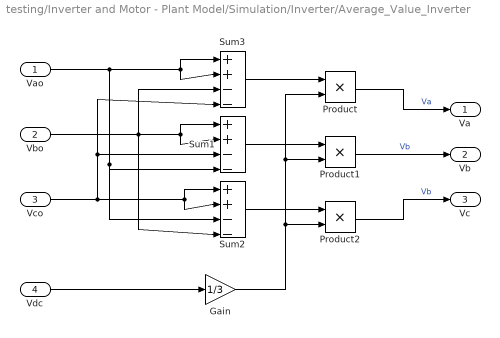
== system testing/Inverter and Motor - Plant Model/Simulation/Inverter/Average_Value_Inverter ==
  Vao : Inport
  Vbo : Inport  Port=2
  Vco : Inport  Port=3
  Vdc : Inport  Port=4
  Gain : Gain  Gain=1/3  RndMeth=Simplest  OutDataTypeStr=Inherit: Same as input
  Product : Product  RndMeth=Simplest  OutDataTypeStr=Inherit: Same as first input
  Product1 : Product  RndMeth=Simplest  OutDataTypeStr=Inherit: Same as first input
  Product2 : Product  RndMeth=Simplest  OutDataTypeStr=Inherit: Same as first input
  Sum1 : Sum  Inputs=|++--  RndMeth=Simplest  OutDataTypeStr=Inherit: Same as first input
  Sum2 : Sum  Inputs=|++--  RndMeth=Simplest  OutDataTypeStr=Inherit: Same as first input
  Sum3 : Sum  Inputs=|++--  RndMeth=Simplest  OutDataTypeStr=Inherit: Same as first input
  Va : Outport  VectorParamsAs1DForOutWhenUnconnected=off
  Vb : Outport  Port=2  VectorParamsAs1DForOutWhenUnconnected=off
  Vc : Outport  Port=3  VectorParamsAs1DForOutWhenUnconnected=off
  wires:
  Product1/1 -> Vb/1  "Vb"
  Gain/1 -> Product/2, Product1/2, Product2/2
  Sum2/1 -> Product2/1
  Vao/1 -> Sum3/1, Sum3/2, Sum1/4, Sum2/3
  Product2/1 -> Vc/1  "Vb"
  Sum1/1 -> Product1/1
  Vdc/1 -> Gain/1
  Sum3/1 -> Product/1
  Product/1 -> Va/1  "Va"
  Vco/1 -> Sum3/4, Sum1/3, Sum2/2, Sum2/1
  Vbo/1 -> Sum1/1, Sum1/2, Sum3/3, Sum2/4

== system testing/Inverter and Motor - Plant Model/Simulation/Sensor_Measurements/Wrap ==
  in : Inport
  Constant2 : Constant  Value=2*pi  OutDataTypeStr=single  SampleTime=-1
  Mod : Math  Operator=mod
  out : Outport  VectorParamsAs1DForOutWhenUnconnected=off
  wires:
  in/1 -> Mod/1
  Constant2/1 -> Mod/2
  Mod/1 -> out/1

== system testing/Hardware Init/Variant Subsystem/Code Generation/Calculate ADC Offset /For Iterator Subsystem ==
  ADC_A_IN0 : c2802xlib/ADC  Priority=20  blkParamProc=C2000_Type4  ADCModule=C  samplingMode=Single sample mode  ADCResolution=12-bit (Single-ended input)  ADC29xResolution=12-bit  ADCMode=Single-ended input  useSOC1=SOC2  useSOC2=SOC0_SOC1  SOCAcquisitionWindow=15  SOCTriggerSource=Software  SOCInterruptTrigger=No ADCINT  Ts=-1  dType=uint16  postInterrupt=off  interruptSel=ADCINT1  ADCINTContinuous=on  endma=off  chdma=1  conv1=ADCINA0  conv2=ADCINA0 and ADCINB0  conv1_Type4=ADCIN2  conv2_Type4=ADCIN0 and ADCIN1
  ADC_B_IN0 : c2802xlib/ADC  Priority=20  blkParamProc=C2000_Type4  ADCModule=B  samplingMode=Single sample mode  ADCResolution=12-bit (Single-ended input)  ADC29xResolution=12-bit  ADCMode=Single-ended input  useSOC1=SOC2  useSOC2=SOC0_SOC1  SOCAcquisitionWindow=15  SOCTriggerSource=Software  SOCInterruptTrigger=No ADCINT  Ts=-1  dType=uint16  postInterrupt=off  interruptSel=ADCINT1  ADCINTContinuous=on  endma=off  chdma=1  conv1=ADCINA0  conv2=ADCINA0 and ADCINB0  conv1_Type4=ADCIN2  conv2_Type4=ADCIN0 and ADCIN1
  For Iterator : ForIterator  IterationLimit=16  IterationVariableDataType=uint16
  If : If  IfExpression=u1 > 8  ShowElse=off
  If Action Subsystem : Subsystem  TreatAsAtomicUnit=on
  Out1 : Outport
  Out2 : Outport  Port=2
  wires:
  For Iterator/1 -> If/1
  ADC_A_IN0/1 -> If Action Subsystem/1(In1)
  ADC_B_IN0/1 -> If Action Subsystem/2(In2)
  If Action Subsystem/1(Out1) -> Out1/1
  If Action Subsystem/2(Out2) -> Out2/1
  If/1 -> If Action Subsystem/Action

== system testing/Hardware Init/Variant Subsystem/Code Generation/Calculate ADC Offset /If Action Subsystem ==
  In1 : Inport
  Action Port : ActionPort  ActionPortLabel=if(u1 > u3 & u1 < u2)
  Data Store Write1 : DataStoreWrite  DataStoreName=IaOffset  IndexOptions=Index vector (dialog)  Indices=1  OutputSizes=1
  wires:
  In1/1 -> Data Store Write1/1

== system testing/Hardware Init/Variant Subsystem/Code Generation/Calculate ADC Offset /If Action Subsystem1 ==
  Action Port : ActionPort  ActionPortLabel=else
  Constant : Constant  Value=inverter.CtSensAOffset  OutDataTypeStr=Inherit: Inherit via back propagation
  Data Store Write1 : DataStoreWrite  DataStoreName=IaOffset  IndexOptions=Index vector (dialog)  Indices=1  OutputSizes=1
  wires:
  Constant/1 -> Data Store Write1/1

== system testing/Hardware Init/Variant Subsystem/Code Generation/Calculate ADC Offset /If Action Subsystem2 ==
  In1 : Inport
  Action Port : ActionPort  ActionPortLabel=if(u1 > u3 & u1 < u2)
  Data Store Write2 : DataStoreWrite  DataStoreName=IbOffset  IndexOptions=Index vector (dialog)  Indices=1  OutputSizes=1
  wires:
  In1/1 -> Data Store Write2/1

== system testing/Hardware Init/Variant Subsystem/Code Generation/Calculate ADC Offset /If Action Subsystem3 ==
  Action Port : ActionPort  ActionPortLabel=else
  Constant1 : Constant  Value=inverter.CtSensBOffset  OutDataTypeStr=Inherit: Inherit via back propagation
  Data Store Write2 : DataStoreWrite  DataStoreName=IbOffset  IndexOptions=Index vector (dialog)  Indices=1  OutputSizes=1
  wires:
  Constant1/1 -> Data Store Write2/1

== system testing/Hardware Init/Variant Subsystem/Code Generation/DRV Enable/ADC Gain Setting ==
  In : Inport
  Enable : EnablePort
  Demux : Demux  Outputs=2
  Display : Display
      settings: Format=hex (Stored Integer)
  Display1 : Display
      settings: Format=hex (Stored Integer)
  SPI Master Transfer : c280xlib/SPI Controller Transfer  SPISelect=SPI_A  ClockPolarity=Rising_edge  ClockPhase=No_delay  SPIModule=uint32(0)  Mode=Master  BusSpeed=uint32(1000000)  FirstBitToTransfer=Most significant bit (MSB)  ClockMode=0  BlockFunction=Transfer  EnableRegisterAddress=off  RegisterAddress=0  OutputDataType=int8  OutputDataLength=1  DataBits=16  UseCustomSSPin=Provided by the SPI peripheral  ActiveLowSSPin=Active low  Pin=61
  SPI Master Transfer1 : c280xlib/SPI Controller Transfer  SPISelect=SPI_A  ClockPolarity=Rising_edge  ClockPhase=No_delay  SPIModule=uint32(0)  Mode=Master  BusSpeed=uint32(1000000)  FirstBitToTransfer=Most significant bit (MSB)  ClockMode=0  BlockFunction=Transfer  EnableRegisterAddress=off  RegisterAddress=0  OutputDataType=int8  OutputDataLength=1  DataBits=16  UseCustomSSPin=Provided by the SPI peripheral  ActiveLowSSPin=Active low  Pin=61
  wires:
  Demux/2 -> SPI Master Transfer1/1
  SPI Master Transfer/1 -> Display/1
  SPI Master Transfer1/1 -> Display1/1
  In/1 -> Demux/1
  Demux/1 -> SPI Master Transfer/1

== system testing/Hardware Init/Variant Subsystem/Code Generation/Calculate ADC Offset /For Iterator Subsystem/If Action Subsystem ==
  In1 : Inport
  In2 : Inport  Port=2
  Action Port : ActionPort  ActionPortLabel=if(u1 > 8)
  Memory : Memory  InheritSampleTime=on
  Memory1 : Memory  InheritSampleTime=on
  Sum : Sum
  Sum1 : Sum
  Out1 : Outport
  Out2 : Outport  Port=2
  wires:
  In1/1 -> Sum/1
  Sum/1 -> Out1/1, Memory/1
  In2/1 -> Sum1/1
  Memory/1 -> Sum/2
  Sum1/1 -> Out2/1, Memory1/1
  Memory1/1 -> Sum1/2

== matlab function testing/MATLAB Function ==
  data: x_pre input; x output; P_pre input; y_true input; uk input; P output
function [x, P] = ekf_pmsm(x_pre, P_pre, y_true, uk)
%#codegen
% Extended Kalman Filter for PMSM mechanical parameter estimation.
%
% Estimates the joint state + parameters of the speed dynamics:
%     wm_dot = -x2*wm + x3*iq - x4*sign(wm)
%
% State vector x = [wm ; x2 ; x3 ; x4]:
%   x1 = wm  : mechanical speed              [rad/s]   (physical state)
%   x2 = Bv/J: viscous-friction / inertia    [1/s]     (parameter, A = -x2)
%   x3 = B   : input gain 3*p*lambda/(2J)    [rad/s/A] (parameter)
%   x4 = Tc/J: Coulomb-friction coefficient  [rad/s^2] (parameter)
%
% Inputs:
%   x_pre  : previous state+parameter estimate [4x1]
%   P_pre  : previous error covariance         [4x4]
%   y_true : measured mechanical speed wm      [rad/s]
%   uk     : control input iq (q-axis current) [A]
%
% Outputs:
%   x : updated estimate  [4x1]  (recover A = -x2)
%   P : updated covariance [4x4]

    % ---- Settings ----
    Ts     = 5e-4;                          % sample time = Ts_speed (10*Ts_pwm)
    Qc_est = 1e-4*diag([1, 0.1, 0.1, 0.001]);  % very low Q on C (x4)   % continuous process-noise weights
    Qd_est = Ts*Qc_est;                     % discretized process noise
    R_est  = 0.01;                          % speed-measurement noise variance
    Ck     = [1 0 0 0];                     % measure speed only
    Dk     = 0;

    % ================= PREDICTION STEP =================
    % Propagate the estimate one step with forward Euler.
    % Parameters (x2,x3,x4) are modelled as constant (zero dynamics),
    % their drift is allowed only through the process noise Qd_est.
    x = x_pre + Ts*[ -x_pre(2)*x_pre(1) + uk*x_pre(3) - x_pre(4)*sign(x_pre(1));
                      0;
                      0;
                      0 ];

    % Jacobian of the dynamics w.r.t. the state (linearization for EKF).
    Ak = eye(4) + Ts*[ -x_pre(2)  -x_pre(1)  uk  -sign(x_pre(1));
                        0          0          0    0;
                        0          0          0    0;
                        0          0          0    0 ];

    % Propagate the covariance.
    P = Ak*P_pre*Ak' + Qd_est;

    % ================= OBSERVATION & UPDATE =================
    % Kalman gain.
    Wk    = P*Ck' / (Ck*P*Ck' + R_est);

    % Innovation: measured minus predicted speed.
    y_est = Ck*x + Dk*uk;
    dely  = y_true - y_est;

    % Correct the estimate and shrink the covariance.
    x = x + Wk*dely;
    P = P - Wk*Ck*P;
end

== matlab function testing/Current Control/Control_System/Closed Loop Control/Current_Controllers/MATLAB Function ==
  data: id input; v_dc output; iq input; wm input
function v_dc = decouple(id, iq, wm)
%#codegen
% Option-B decoupling feedforward for surface PMSM (Teknic 2310P)
% wm = mechanical speed [rad/s], id/iq = measured dq currents [A]

    % --- Motor parameters ---
    Ld     = 2.0e-4;    % d-axis inductance [H]
    Lq     = 2.0e-4;    % q-axis inductance [H]
    lambda = 0.0064;    % PM flux linkage [Wb]
    p      = 4;         % pole pairs

    % --- Electrical speed ---
    we = p * wm;        % electrical angular speed [rad/s]

    % --- Decoupling feedforward (adds back the cancelled coupling + back-EMF) ---
    vd_dc = -we * Lq * iq;
    vq_dc =  we * Ld * id + we * lambda;

    v_dc = [vd_dc; vq_dc];   % 2x1: [Vd_decouple; Vq_decouple]
end

== matlab function testing/MATLAB Function1 ==
  data: A_est input; Ks output; B_est input; Kis output
function [Ks, Kis] = adaptive_gains(A_est, B_est)
    wc = 50;                    % speed-loop bandwidth
    p1 = wc;  p2 = 1.2*wc;      % desired poles
    Ts_speed = 5e-4;            % speed-loop sample time

    A_s = -A_est;               % EKF estimates -A_s, so negate
    B_safe = min(B_est, 1000);  % avoid division by zero

    Ks  = (p1 + p2 + A_s) / B_safe;
    Kis = (p1 * p2) / B_safe * Ts_speed;   % output Ki*Ts for the PI block
end

== matlab function testing/MATLAB Function2 ==
  data: P input; trP output
function trP = param_trace(P)
%#codegen
% Sum of the parameter variances (diagonal entries for A, B, C).
% P is the 4x4 EKF covariance; states are [wm, A, B, C] at indices 1..4.
% We ignore P(1,1) (the speed state) and sum the parameter diagonal.
    trP = P(2,2) + P(3,3) + P(4,4);
end
